simulink subsystem "energy_meter"  (R2025b)
settings: Solver=VariableStepAuto  StartTime=0.0  StopTime=10.0  RelTol=1e-3
undefined symbols (not defined in the file): DiscIntNeverNeededParam
settings Model: Creator=lenovo  LastModifiedBy=lenovo

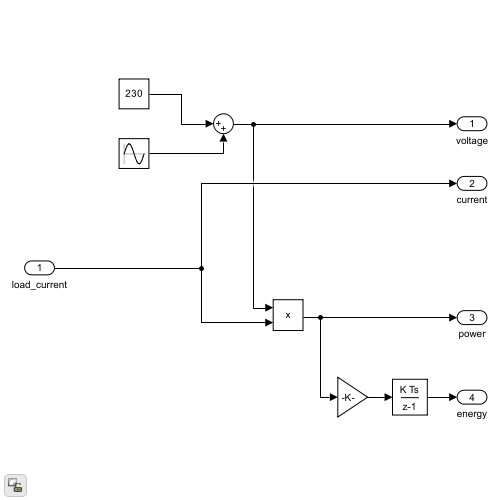
[thumbnail: Simulink's stored preview of the top-level diagram]
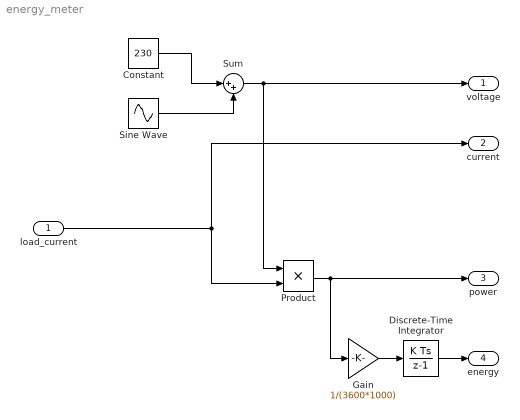
== system energy_meter ==
  load_current : Inport
  Constant : Constant  Value=230
  Discrete-Time Integrator : DiscreteIntegrator  SampleTime=-1  ICPrevOutput=DiscIntNeverNeededParam  ICPrevScaledInput=DiscIntNeverNeededParam
  Gain : Gain  Gain=1/(3600*1000)
  Product : Product
  Sine Wave : Sin  Amplitude=10  Frequency=(2*pi)/86400  SampleTime=0
  Sum : Sum  Inputs=|++
  voltage : Outport
  current : Outport  Port=2
  power : Outport  Port=3
  energy : Outport  Port=4
  wires:
  Constant/1 -> Sum/1
  Sine Wave/1 -> Sum/2
  Sum/1 -> Product/1, voltage/1
  load_current/1 -> current/1, Product/2
  Product/1 -> Gain/1, power/1
  Discrete-Time Integrator/1 -> energy/1
  Gain/1 -> Discrete-Time Integrator/1
